simulink subsystem "cascaded_pid_controller"  (R2026a)
settings: Solver=VariableStepAuto
undefined symbols (not defined in the file): DiscIntNeverNeededParam, dspblkCoreblockFVToolHelper, FF_maneuvers, gcbh, I, P, RSFF_maneuvers, S, T
libraries: slpidlib x3, simulink x1
PreSaveFcn:
  | defaultToFileBlockNames(bdroot);
settings Model: Creator=kjhaydon  LastModifiedBy=kjhaydon

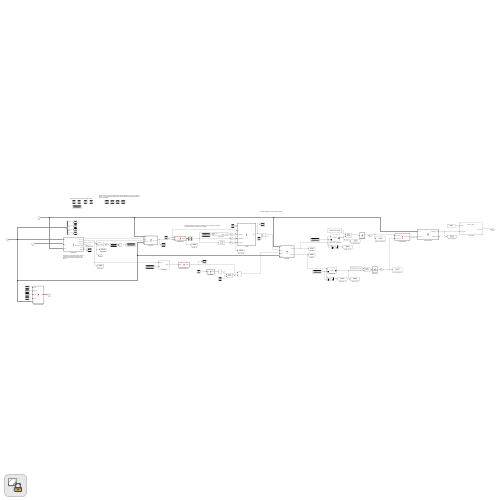
[thumbnail: Simulink's stored preview of the top-level diagram]
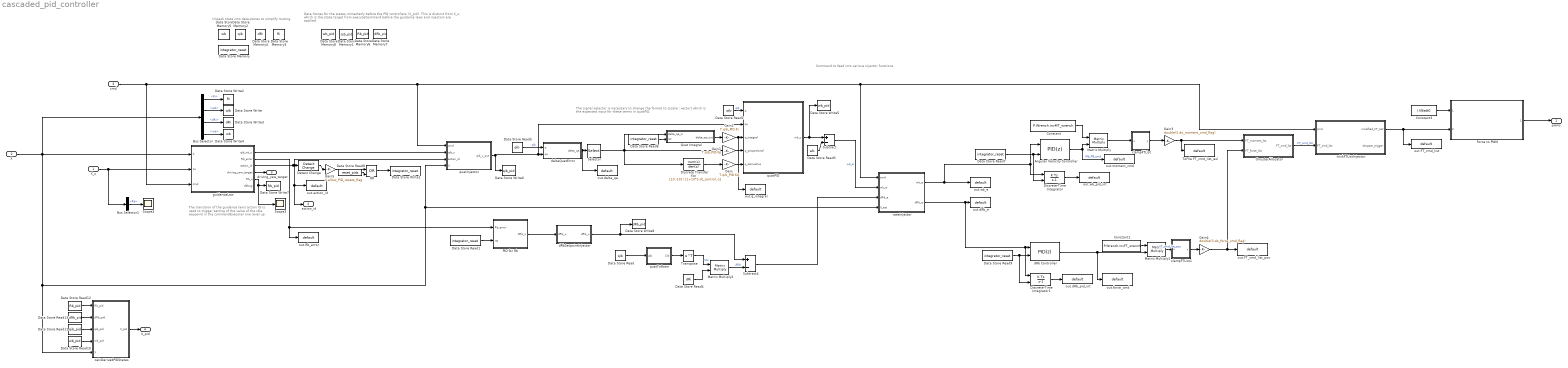
== system cascaded_pid_controller ==
  note: Data Stores for the states immediatly before the PID controllers (X_pid). This is distinct from X_u, which is the state target from executeCommand before the guidance laws and injectors are applied.
  note: Unpack state into data-stores to simplify routing.
  note: The transition of the guidance law's action ID is used to trigger setting of the value of the idle waypoint in the commandExecuter one level up.
  note: The signal selector is necessary to change the format to [scalar; vector] which
      | is the expected input for these terms in quatPID.
  note: Command to feed into various injector functions.
  X_u : Inport  SampleTime=S.dt_control
  X : Inport  Port=2  SampleTime=S.dt_control
  cmd : Inport  Port=3  SampleTime=S.dt_control
  Angular Velocity Controller : slpidlib/PID Controller  Controller=PID  Form=Parallel  TimeDomain=Discrete-time  UseExternalTs=off  SampleTime=-1  IntegratorMethod=Forward Euler  FilterMethod=Forward Euler  ControllerParametersSource=internal  P=T.wb_PID.Kp  I=T.wb_PID.Ki  UseKiTs=off  D=T.wb_PID.Kd  UseExternalDerivativeSource=off  N=T.wb_PID.N  UseFilter=on  TunerSelectOption=Transfer Function Based (PID Tuner App)  InitialConditionSource=internal  InitialConditionForIntegrator=0  InitialConditionForFilter=0  DifferentiatorICPrevScaledInput=0  ExternalReset=rising  TrackingMode=off  Kt=1  LimitOutput=on  SatLimitsSource=internal  UpperSaturationLimit=T.wb_PID.output_sat  LowerSaturationLimit=-T.wb_PID.output_sat  LinearizeAsGain=on  AntiWindupMode=clamping  Kb=1  LimitIntegrator=on  UpperIntegratorSaturationLimit=T.wb_PID.int_sat  LowerIntegratorSaturationLimit=-T.wb_PID.int_sat  POutMin=[]  POutMax=[]  IOutMin=[]  IOutMax=[]  DOutMin=[]  DOutMax=[]  NOutMin=[]  NOutMax=[]  SumOutMin=[]  SumOutMax=[]  SaturationOutMin=[]  SaturationOutMax=[]  PParamMin=[]  PParamMax=[]  IParamMin=[]  IParamMax=[]  DParamMin=[]  DParamMax=[]  NParamMin=[]  NParamMax=[]  KbParamMin=[]  KbParamMax=[]  KtParamMin=[]  KtParamMax=[]  KbOutMin=[]  KbOutMax=[]  KtOutMin=[]  KtOutMax=[]  IntegratorOutMin=[]  IntegratorOutMax=[]  FilterOutMin=[]  FilterOutMax=[]  SumI1OutMin=[]  SumI1OutMax=[]  SumI2OutMin=[]  SumI2OutMax=[]  SumI3OutMin=[]  SumI3OutMax=[]  SumI4OutMin=[]  SumI4OutMax=[]  SumDOutMin=[]  SumDOutMax=[]  DifferentiatorOutMin=[]  DifferentiatorOutMax=[]  FilterDiffOutCoefMin=[]  FilterDiffOutCoefMax=[]  ReciprocalOutMin=[]  ReciprocalOutMax=[]  SumDenOutMin=[]  SumDenOutMax=[]  SumNumOutMin=[]  SumNumOutMax=[]  DivideOutMin=[]  DivideOutMax=[]  UdiffTsProdOutMin=[]  UdiffTsProdOutMax=[]  NTsProdOutMin=[]  NTsProdOutMax=[]  UintegralTsProdOutMin=[]  UintegralTsProdOutMax=[]  UngainTsProdOutMin=[]  UngainTsProdOutMax=[]  ClampingZeroOutDataTypeStr=Inherit: Inherit via back propagation  ClampingZeroOutMin=[]  ClampingZeroOutMax=[]  FilterDenConstantOutDataTypeStr=Inherit: Inherit via back propagation  FilterDenConstantOutMin=[]  FilterDenConstantOutMax=[]  PCopyOutDataTypeStr=Inherit: Inherit via back propagation  PCopyOutMin=[]  PCopyOutMax=[]  NCopyOutDataTypeStr=Inherit: Inherit via back propagation  NCopyOutMin=[]  NCopyOutMax=[]  IntegratorContinuousStateAttributes=''  IntegratorStateMustResolveToSignalObject=off  IntegratorRTWStateStorageClass=Auto  FilterContinuousStateAttributes=''  FilterStateMustResolveToSignalObject=off  FilterRTWStateStorageClass=Auto  ParallelPVariant=InternalParameters  IdealPVariant=Disabled  IVariant=InternalParameters  DVariant=InternalParameters  IntegratorVariant=Discrete  SatVariant=Enabled  AWVariant=DiscClampingParallel  PCopyVariant=Disabled  TRVariant=Disabled  FdbkBlocksVariant=Forward  IdealPFdbkVariant=Disabled  SatFdbkVariant=Disabled  DerivativeFilterVariant=ForwardEulerFilter  NVariant=InternalParameters  NCopyVariant=Disabled  FilterICVariant=InternalICsFilter  IntegratorICVariant=InternalICs  ExternalResetVariant=ExternalReset  TRSumVariant=Passthrough  SumFdbkVariant=Disabled  SumVariant=Sum_PID  TsampFilterVariant=InternalTs  TsampNgainVariant=Passthrough  TsampIntegralVariant=Disabled_SignalSpec  ExternalSaturationOutDataTypeStr=Inherit: Same as second input  DerivativeSourceVariant=ErrorSignal  PreIntVariant=InternalPreInt
  Bus Selector : BusSelector  OutputSignals=Ri,qib,dRi,wb
  Bus Selector1 : BusSelector  OutputSignals=Rb
  Constant : Constant  Value=P.Wrench.invMT_wrench
  Constant1 : Constant  Value=P.Wrench.invFT_wrench
  Constant3 : Constant  Value=I.VBatt0
  Data Store Memory : DataStoreMemory  DataStoreName=integrator_reset  WriteAfterWriteMsg=warning  ShowAdditionalParam=off
  Data Store Memory1 : DataStoreMemory  DataStoreName=qib_pid  WriteAfterWriteMsg=warning  InitialValue=[0 0 0 1]'  ShowAdditionalParam=off
  Data Store Memory2 : DataStoreMemory  DataStoreName=qib  WriteAfterWriteMsg=warning  InitialValue=[0 0 0 1]'  ShowAdditionalParam=off
  Data Store Memory3 : DataStoreMemory  DataStoreName=Ri  WriteAfterWriteMsg=warning  InitialValue=[0 0 0]'  ShowAdditionalParam=off
  Data Store Memory4 : DataStoreMemory  DataStoreName=dRi  WriteAfterWriteMsg=warning  InitialValue=[0 0 0]'  ShowAdditionalParam=off
  Data Store Memory5 : DataStoreMemory  DataStoreName=wb  WriteAfterWriteMsg=warning  InitialValue=[0 0 0]'  ShowAdditionalParam=off
  Data Store Memory6 : DataStoreMemory  DataStoreName=Rb_pid  WriteAfterWriteMsg=warning  InitialValue=[0 0 0]'  ShowAdditionalParam=off
  Data Store Memory7 : DataStoreMemory  DataStoreName=dRb_pid  WriteAfterWriteMsg=warning  InitialValue=[0 0 0]'  ShowAdditionalParam=off
  Data Store Memory8 : DataStoreMemory  DataStoreName=wb_pid  WriteAfterWriteMsg=warning  InitialValue=[0 0 0]'  ShowAdditionalParam=off
  Data Store Read : DataStoreRead  DataStoreName=qib  IndexOptions=Index vector (dialog)  Indices=1  OutputSizes=1
  Data Store Read{1,6..7,9} (4 alike) : DataStoreRead  DataStoreName=integrator_reset  IndexOptions=Index vector (dialog)  Indices=1  OutputSizes=1
  Data Store Read10 : DataStoreRead  DataStoreName=wb_pid  IndexOptions=Index vector (dialog)  Indices=1  OutputSizes=1
  Data Store Read11 : DataStoreRead  DataStoreName=qib_pid  IndexOptions=Index vector (dialog)  Indices=1  OutputSizes=1
  Data Store Read12 : DataStoreRead  DataStoreName=Rb_pid  IndexOptions=Index vector (dialog)  Indices=1  OutputSizes=1
  Data Store Read13 : DataStoreRead  DataStoreName=dRb_pid  IndexOptions=Index vector (dialog)  Indices=1  OutputSizes=1
  Data Store Read2 : DataStoreRead  DataStoreName=qib  IndexOptions=Index vector (dialog)  Indices=1  OutputSizes=1
  Data Store Read3 : DataStoreRead  DataStoreName=wb  IndexOptions=Index vector (dialog)  Indices=1  OutputSizes=1
  Data Store Read4 : DataStoreRead  DataStoreName=dRi  IndexOptions=Index vector (dialog)  Indices=1  OutputSizes=1
  Data Store Read5 : DataStoreRead  DataStoreName=qib  IndexOptions=Index vector (dialog)  Indices=1  OutputSizes=1
  Data Store Read8 : DataStoreRead  DataStoreName=reset_pids  IndexOptions=Index vector (dialog)  Indices=1  OutputSizes=1
  Data Store Write : DataStoreWrite  DataStoreName=qib  IndexOptions=Index vector (dialog)  Indices=1  OutputSizes=1
  Data Store Write1 : DataStoreWrite  DataStoreName=integrator_reset  IndexOptions=Index vector (dialog)  Indices=1  OutputSizes=1
  Data Store Write2 : DataStoreWrite  DataStoreName=Ri  IndexOptions=Index vector (dialog)  Indices=1  OutputSizes=1
  Data Store Write3 : DataStoreWrite  DataStoreName=dRi  IndexOptions=Index vector (dialog)  Indices=1  OutputSizes=1
  Data Store Write4 : DataStoreWrite  DataStoreName=wb  IndexOptions=Index vector (dialog)  Indices=1  OutputSizes=1
  Data Store Write5 : DataStoreWrite  DataStoreName=wb_pid  IndexOptions=Index vector (dialog)  Indices=1  OutputSizes=1
  Data Store Write6 : DataStoreWrite  DataStoreName=qib_pid  IndexOptions=Index vector (dialog)  Indices=1  OutputSizes=1
  Data Store Write7 : DataStoreWrite  DataStoreName=Rb_pid  IndexOptions=Index vector (dialog)  Indices=1  OutputSizes=1
  Data Store Write8 : DataStoreWrite  DataStoreName=dRb_pid  IndexOptions=Index vector (dialog)  Indices=1  OutputSizes=1
  Detect Change : simulink/Logic and Bit Operations/Detect Change  vinit=0  OutDataTypeStr=boolean
  Discrete Transfer Fcn : DiscreteTransferFcn  LoadFcn=dspblkCoreblockFVToolHelper(gcbh,'load');  Numerator=[10,-10]  Denominator=[1+10*S.dt_control,-1]
      settings: CopyFcn=dspblkCoreblockFVToolHelper(gcbh,'copy');  DeleteFcn=dspblkCoreblockFVToolHelper(gcbh,'close');  ModelCloseFcn=dspblkCoreblockFVToolHelper(gcbh,'close');  PreSaveFcn=dspblkCoreblockFVToolHelper(gcbh,'presave');  PostSaveFcn=dspblkCoreblockFVToolHelper(gcbh,'postsave');  CloseFcn=dspblkCoreblockFVToolHelper(gcbh,'close');
  Discrete-Time Integrator : DiscreteIntegrator  gainval=T.wb_PID.Ki  ExternalReset=rising  InitialCondition=[0;0;0]  SampleTime=S.dt_control  LimitOutput=on  UpperSaturationLimit=T.wb_PID.int_sat  LowerSaturationLimit=-T.wb_PID.int_sat  ICPrevOutput=DiscIntNeverNeededParam  ICPrevScaledInput=DiscIntNeverNeededParam
  Discrete-Time Integrator1 : DiscreteIntegrator  gainval=T.dRb_PID.Ki  ExternalReset=rising  InitialCondition=[0;0;0]  SampleTime=S.dt_control  LimitOutput=on  UpperSaturationLimit=T.dRb_PID.int_sat  LowerSaturationLimit=-T.dRb_PID.int_sat  ICPrevOutput=DiscIntNeverNeededParam  ICPrevScaledInput=DiscIntNeverNeededParam
  Force to PWM : Subsystem  ReferencedSubsystem=force_to_pwm
  Gain : Gain  Gain=T.qib_PID.Kd
  Gain1 : Gain  Gain=T.qib_PID.Kp
  Gain2 : Gain  Gain=T.qib_PID.Ki
  Gain3 : Gain  Gain=double(S.do_moment_cmd_flag)
  Gain4 : Gain  Gain=double(S.do_force_cmd_flag)
  Gain5 : Gain  Gain=S.allow_PID_resets_flag
  Matrix Multiply : Product  Multiplication=Matrix(*)
  Matrix Multiply1 : Product  Multiplication=Matrix(*)
  Matrix Multiply3 : Product  Multiplication=Matrix(*)
  OR : Logic  Operator=OR  IconShape=distinctive  AllPortsSameDT=off  OutDataTypeStr=boolean
  PID for Rb : Subsystem
  Quat Integral : Subsystem
  Scope3 : Scope
      settings: ActiveDisplayYMinimum=-2.6644023015259384  ActiveDisplayYMaximum=2.5944913455232195  DataLoggingVariableName=ScopeData6
  Scope4 : Scope
      settings: ActiveDisplayYMinimum=-6.74848704493326  ActiveDisplayYMaximum=15.916420433675906  DataLoggingVariableName=ScopeData7
  Selector : Selector  InputPortWidth=4  IndexOptions=Index vector (dialog)  Indices=[4 1 2 3]  OutputSizes=1
  Subtract : Sum  Inputs=+-
  Subtract4 : Sum  Inputs=+-
  ToFIle FT_cmd_list_eul : ToFile  Filename=default  MatrixName=FT_cmd_list_eul  SaveFormat=Timeseries  SampleTime=S.dt_data
  Transpose : Math  Operator=transpose
  calcDerivedPIDStates : MATLAB Function  TreatAsAtomicUnit=on
  clampFTList : MATLAB Function  TreatAsAtomicUnit=on
  clampFTList1 : MATLAB Function  TreatAsAtomicUnit=on
  dRb Controller : slpidlib/PID Controller  Controller=PID  Form=Parallel  TimeDomain=Discrete-time  UseExternalTs=off  SampleTime=-1  IntegratorMethod=Forward Euler  FilterMethod=Forward Euler  ControllerParametersSource=internal  P=T.dRb_PID.Kp  I=T.dRb_PID.Ki  UseKiTs=off  D=T.dRb_PID.Kd  UseExternalDerivativeSource=off  N=T.dRb_PID.N  UseFilter=on  TunerSelectOption=Transfer Function Based (PID Tuner App)  InitialConditionSource=internal  InitialConditionForIntegrator=0  InitialConditionForFilter=0  DifferentiatorICPrevScaledInput=0  ExternalReset=rising  TrackingMode=off  Kt=1  LimitOutput=on  SatLimitsSource=internal  UpperSaturationLimit=T.dRb_PID.output_sat  LowerSaturationLimit=-T.dRb_PID.output_sat  LinearizeAsGain=on  AntiWindupMode=clamping  Kb=1  LimitIntegrator=on  UpperIntegratorSaturationLimit=T.dRb_PID.int_sat  LowerIntegratorSaturationLimit=-T.dRb_PID.int_sat  POutMin=[]  POutMax=[]  IOutMin=[]  IOutMax=[]  DOutMin=[]  DOutMax=[]  NOutMin=[]  NOutMax=[]  SumOutMin=[]  SumOutMax=[]  SaturationOutMin=[]  SaturationOutMax=[]  PParamMin=[]  PParamMax=[]  IParamMin=[]  IParamMax=[]  DParamMin=[]  DParamMax=[]  NParamMin=[]  NParamMax=[]  KbParamMin=[]  KbParamMax=[]  KtParamMin=[]  KtParamMax=[]  KbOutMin=[]  KbOutMax=[]  KtOutMin=[]  KtOutMax=[]  IntegratorOutMin=[]  IntegratorOutMax=[]  FilterOutMin=[]  FilterOutMax=[]  SumI1OutMin=[]  SumI1OutMax=[]  SumI2OutMin=[]  SumI2OutMax=[]  SumI3OutMin=[]  SumI3OutMax=[]  SumI4OutMin=[]  SumI4OutMax=[]  SumDOutMin=[]  SumDOutMax=[]  DifferentiatorOutMin=[]  DifferentiatorOutMax=[]  FilterDiffOutCoefMin=[]  FilterDiffOutCoefMax=[]  ReciprocalOutMin=[]  ReciprocalOutMax=[]  SumDenOutMin=[]  SumDenOutMax=[]  SumNumOutMin=[]  SumNumOutMax=[]  DivideOutMin=[]  DivideOutMax=[]  UdiffTsProdOutMin=[]  UdiffTsProdOutMax=[]  NTsProdOutMin=[]  NTsProdOutMax=[]  UintegralTsProdOutMin=[]  UintegralTsProdOutMax=[]  UngainTsProdOutMin=[]  UngainTsProdOutMax=[]  ClampingZeroOutDataTypeStr=Inherit: Inherit via back propagation  ClampingZeroOutMin=[]  ClampingZeroOutMax=[]  FilterDenConstantOutDataTypeStr=Inherit: Inherit via back propagation  FilterDenConstantOutMin=[]  FilterDenConstantOutMax=[]  PCopyOutDataTypeStr=Inherit: Inherit via back propagation  PCopyOutMin=[]  PCopyOutMax=[]  NCopyOutDataTypeStr=Inherit: Inherit via back propagation  NCopyOutMin=[]  NCopyOutMax=[]  IntegratorContinuousStateAttributes=''  IntegratorStateMustResolveToSignalObject=off  IntegratorRTWStateStorageClass=Auto  FilterContinuousStateAttributes=''  FilterStateMustResolveToSignalObject=off  FilterRTWStateStorageClass=Auto  ParallelPVariant=InternalParameters  IdealPVariant=Disabled  IVariant=InternalParameters  DVariant=InternalParameters  IntegratorVariant=Discrete  SatVariant=Enabled  AWVariant=DiscClampingParallel  PCopyVariant=Disabled  TRVariant=Disabled  FdbkBlocksVariant=Forward  IdealPFdbkVariant=Disabled  SatFdbkVariant=Disabled  DerivativeFilterVariant=ForwardEulerFilter  NVariant=InternalParameters  NCopyVariant=Disabled  FilterICVariant=InternalICsFilter  IntegratorICVariant=InternalICs  ExternalResetVariant=ExternalReset  TRSumVariant=Passthrough  SumFdbkVariant=Disabled  SumVariant=Sum_PID  TsampFilterVariant=InternalTs  TsampNgainVariant=Passthrough  TsampIntegralVariant=Disabled_SignalSpec  ExternalSaturationOutDataTypeStr=Inherit: Same as second input  DerivativeSourceVariant=ErrorSignal  PreIntVariant=InternalPreInt
  dRbSetpointInjector : MATLAB Function  TreatAsAtomicUnit=on
  deltaQuatError : MATLAB Function  TreatAsAtomicUnit=on
  guidanceLaw : MATLAB Function  TreatAsAtomicUnit=on
  out.FT_cmd_list : ToFile  Filename=default  MatrixName=FT_cmd_list  SaveFormat=Timeseries  SampleTime=S.dt_data
  out.FT_cmd_list_pos : ToFile  Filename=default  MatrixName=FT_cmd_list_pos  SaveFormat=Timeseries  SampleTime=S.dt_data
  out.Rb_error : ToFile  Filename=default  MatrixName=Rb_e  SaveFormat=Timeseries  SampleTime=S.dt_data
  out.action_id : ToFile  Filename=default  MatrixName=action_id  SaveFormat=Timeseries  SampleTime=S.dt_control
  out.dRb_e : ToFile  Filename=default  MatrixName=dRb_e  SaveFormat=Timeseries  SampleTime=S.dt_data
  out.dRb_pid_int : ToFile  Filename=default  MatrixName=dRb_pid_int  SaveFormat=Timeseries  SampleTime=S.dt_data
  out.delta_qe : ToFile  Filename=default  MatrixName=qib_e  SaveFormat=Timeseries  SampleTime=S.dt_data
  out.force_cmd : ToFile  Filename=default  MatrixName=force_cmd  SaveFormat=Timeseries  SampleTime=S.dt_data
  out.moment_cmd : ToFile  Filename=default  MatrixName=moment_cmd  SaveFormat=Timeseries  SampleTime=S.dt_data
  out.q_integral : ToFile  Filename=default  MatrixName=qib_integrator  SaveFormat=Timeseries  SampleTime=S.dt_data
  out.wb_e : ToFile  Filename=default  MatrixName=wb_e  SaveFormat=Timeseries  SampleTime=S.dt_data
  out.wb_pid_int : ToFile  Filename=default  MatrixName=wb_pid_int  SaveFormat=Timeseries  SampleTime=S.dt_data
  quatInjector : MATLAB Function  TreatAsAtomicUnit=on
  quatPID : MATLAB Function  TreatAsAtomicUnit=on
  quatToRotm : MATLAB Function  TreatAsAtomicUnit=on
  rateInjector : MATLAB Function  TreatAsAtomicUnit=on
  thrusterAllocator : MATLAB Function  TreatAsAtomicUnit=on
  trickFTListInjector : MATLAB Function  TreatAsAtomicUnit=on
  pwms : Outport
  action_id : Outport  Port=2
  driving_yaw_target : Outport  Port=3
  X_pid : Outport  Port=4
  wires:
  calcDerivedPIDStates/1(X_pid) -> X_pid/1
  dRb Controller/1 -> out.force_cmd/1, Matrix Multiply1/2
  guidanceLaw/5(Rb_u) -> Data Store Write7/1, Scope3/1
  Gain4/1 -> thrusterAllocator/2(FT_force_list), out.FT_cmd_list_pos/1
  quatInjector/1(qib_u_out) -> quatPID/2(qu), deltaQuatError/2(qu), Data Store Write6/1
  rateInjector/2(dRb_e) -> dRb Controller/1, Discrete-Time Integrator1/1, out.dRb_e/1
  Subtract4/1 -> rateInjector/3("dRb_e ")
  rateInjector/1(wb_e) -> Angular Velocity Controller/1, Discrete-Time Integrator/1, out.wb_e/1
  Subtract/1 -> rateInjector/2("wb_e ")  "wb_e"
  Data Store Read6/1 -> Quat Integral/2(rst)
  trickFTListInjector/1(modified_FT_List) -> Force to PWM/2, out.FT_cmd_list/1
  cmd/1 -> guidanceLaw/3(cmd), trickFTListInjector/1(cmd), rateInjector/1(cmd), quatInjector/1(cmd)
  thrusterAllocator/1(FT_cmd_list) -> trickFTListInjector/2(FT_cmd_list)  "FT_cmd_list"
  Force to PWM/1 -> pwms/1
  guidanceLaw/3(action_id) -> Detect Change/1, quatInjector/3(action_id), out.action_id/1, action_id/1
  guidanceLaw/1(qib_int_u) -> quatInjector/2(qib_u)
  X_u/1 -> guidanceLaw/2(Xu), Bus Selector1/1
  deltaQuatError/1(delta_qe) -> Selector/1, out.delta_qe/1
  Gain2/1 -> quatPID/3(q_integral), out.q_integral/1
  Gain1/1 -> quatPID/4(q_proportional)
  Gain/1 -> quatPID/5(q_derivative)
  quatPID/1(wb_u) -> Data Store Write5/1, Subtract/1
  Angular Velocity Controller/1 -> out.moment_cmd/1, Matrix Multiply/2  "Mb_FB_cmd"
  Constant/1 -> Matrix Multiply/1
  Constant3/1 -> Force to PWM/1
  Matrix Multiply/1 -> clampFTList/1(u)
  Constant1/1 -> Matrix Multiply1/1
  Matrix Multiply1/1 -> clampFTList1/1(u)  "FT_cmd_list_pos"
  Data Store Read/1 -> quatToRotm/1(qib)
  quatToRotm/1(Cib) -> Transpose/1
  Transpose/1 -> Matrix Multiply3/1  "Cbi"
  Matrix Multiply3/1 -> Subtract4/2  "dRb"
  Data Store Read4/1 -> Matrix Multiply3/2
  Data Store Read3/1 -> Subtract/2
  Data Store Read2/1 -> quatPID/1(q)  "qib"
  Data Store Read5/1 -> deltaQuatError/1(q)  "qib"
  Selector/1 -> Discrete Transfer Fcn/1, Gain1/1, Quat Integral/1(delta_qe_in)
  Quat Integral/1(delta_qe_out) -> Gain2/1
  Discrete Transfer Fcn/1 -> Gain/1
  guidanceLaw/2(Rb_error) -> out.Rb_error/1, PID for Rb/1(Rb_error)
  PID for Rb/1(dRb_u) -> dRbSetpointInjector/1("dRb_u ")
  guidanceLaw/4(driving_yaw_target) -> driving_yaw_target/1
  Bus Selector/1 -> Data Store Write2/1  "<Ri>"
  Bus Selector/2 -> Data Store Write/1  "<qib>"
  Bus Selector/3 -> Data Store Write3/1  "<dRi>"
  Bus Selector/4 -> Data Store Write4/1  "<wb>"
  Data Store Read7/1 -> Discrete-Time Integrator/2, Angular Velocity Controller/2
  Data Store Read9/1 -> Discrete-Time Integrator1/2, dRb Controller/2
  Discrete-Time Integrator/1 -> out.wb_pid_int/1
  Detect Change/1 -> Gain5/1
  dRbSetpointInjector/1(dRb_u) -> Data Store Write8/1, Subtract4/1
  Discrete-Time Integrator1/1 -> out.dRb_pid_int/1
  Gain3/1 -> thrusterAllocator/1(FT_moment_list), ToFIle FT_cmd_list_eul/1
  Gain5/1 -> OR/1
  OR/1 -> Data Store Write1/1
  Data Store Read8/1 -> OR/2
  Data Store Read11/1 -> calcDerivedPIDStates/3(qib_pid)
  X/1 -> guidanceLaw/1(X), Bus Selector/1, quatInjector/4(X), rateInjector/4(X_est), calcDerivedPIDStates/5(X)
  Data Store Read12/1 -> calcDerivedPIDStates/1(Rb_pid)
  Data Store Read10/1 -> calcDerivedPIDStates/4(wb_pid)
  Data Store Read13/1 -> calcDerivedPIDStates/2(dRb_pid)
  clampFTList/1(y) -> Gain3/1
  clampFTList1/1(y) -> Gain4/1
  Data Store Read1/1 -> PID for Rb/2(rst)
  Bus Selector1/1 -> Scope4/1  "<Rb>"

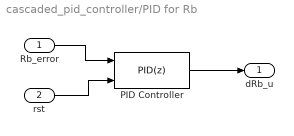
== system cascaded_pid_controller/PID for Rb ==
  Rb_error : Inport
  rst : Inport  Port=2
  PID Controller : slpidlib/PID Controller  Controller=PID  Form=Parallel  TimeDomain=Discrete-time  UseExternalTs=off  SampleTime=-1  IntegratorMethod=Forward Euler  FilterMethod=Forward Euler  ControllerParametersSource=internal  P=T.Rb_PID.Kp  I=T.Rb_PID.Ki  UseKiTs=off  D=T.Rb_PID.Kd  UseExternalDerivativeSource=off  N=T.Rb_PID.N  UseFilter=on  TunerSelectOption=Transfer Function Based (PID Tuner App)  InitialConditionSource=internal  InitialConditionForIntegrator=0  InitialConditionForFilter=0  DifferentiatorICPrevScaledInput=0  ExternalReset=rising  TrackingMode=off  Kt=1  LimitOutput=on  SatLimitsSource=internal  UpperSaturationLimit=T.Rb_PID.output_sat  LowerSaturationLimit=-T.Rb_PID.output_sat  LinearizeAsGain=on  AntiWindupMode=clamping  Kb=1  LimitIntegrator=on  UpperIntegratorSaturationLimit=T.Rb_PID.int_sat  LowerIntegratorSaturationLimit=-T.Rb_PID.int_sat  POutMin=[]  POutMax=[]  IOutMin=[]  IOutMax=[]  DOutMin=[]  DOutMax=[]  NOutMin=[]  NOutMax=[]  SumOutMin=[]  SumOutMax=[]  SaturationOutMin=[]  SaturationOutMax=[]  PParamMin=[]  PParamMax=[]  IParamMin=[]  IParamMax=[]  DParamMin=[]  DParamMax=[]  NParamMin=[]  NParamMax=[]  KbParamMin=[]  KbParamMax=[]  KtParamMin=[]  KtParamMax=[]  KbOutMin=[]  KbOutMax=[]  KtOutMin=[]  KtOutMax=[]  IntegratorOutMin=[]  IntegratorOutMax=[]  FilterOutMin=[]  FilterOutMax=[]  SumI1OutMin=[]  SumI1OutMax=[]  SumI2OutMin=[]  SumI2OutMax=[]  SumI3OutMin=[]  SumI3OutMax=[]  SumI4OutMin=[]  SumI4OutMax=[]  SumDOutMin=[]  SumDOutMax=[]  DifferentiatorOutMin=[]  DifferentiatorOutMax=[]  FilterDiffOutCoefMin=[]  FilterDiffOutCoefMax=[]  ReciprocalOutMin=[]  ReciprocalOutMax=[]  SumDenOutMin=[]  SumDenOutMax=[]  SumNumOutMin=[]  SumNumOutMax=[]  DivideOutMin=[]  DivideOutMax=[]  UdiffTsProdOutMin=[]  UdiffTsProdOutMax=[]  NTsProdOutMin=[]  NTsProdOutMax=[]  UintegralTsProdOutMin=[]  UintegralTsProdOutMax=[]  UngainTsProdOutMin=[]  UngainTsProdOutMax=[]  ClampingZeroOutDataTypeStr=Inherit: Inherit via back propagation  ClampingZeroOutMin=[]  ClampingZeroOutMax=[]  FilterDenConstantOutDataTypeStr=Inherit: Inherit via back propagation  FilterDenConstantOutMin=[]  FilterDenConstantOutMax=[]  PCopyOutDataTypeStr=Inherit: Inherit via back propagation  PCopyOutMin=[]  PCopyOutMax=[]  NCopyOutDataTypeStr=Inherit: Inherit via back propagation  NCopyOutMin=[]  NCopyOutMax=[]  IntegratorContinuousStateAttributes=''  IntegratorStateMustResolveToSignalObject=off  IntegratorRTWStateStorageClass=Auto  FilterContinuousStateAttributes=''  FilterStateMustResolveToSignalObject=off  FilterRTWStateStorageClass=Auto  ParallelPVariant=InternalParameters  IdealPVariant=Disabled  IVariant=InternalParameters  DVariant=InternalParameters  IntegratorVariant=Discrete  SatVariant=Enabled  AWVariant=DiscClampingParallel  PCopyVariant=Disabled  TRVariant=Disabled  FdbkBlocksVariant=Forward  IdealPFdbkVariant=Disabled  SatFdbkVariant=Disabled  DerivativeFilterVariant=ForwardEulerFilter  NVariant=InternalParameters  NCopyVariant=Disabled  FilterICVariant=InternalICsFilter  IntegratorICVariant=InternalICs  ExternalResetVariant=ExternalReset  TRSumVariant=Passthrough  SumFdbkVariant=Disabled  SumVariant=Sum_PID  TsampFilterVariant=InternalTs  TsampNgainVariant=Passthrough  TsampIntegralVariant=Disabled_SignalSpec  ExternalSaturationOutDataTypeStr=Inherit: Same as second input  DerivativeSourceVariant=ErrorSignal  PreIntVariant=InternalPreInt
  dRb_u : Outport
  wires:
  rst/1 -> PID Controller/2
  PID Controller/1 -> dRb_u/1
  Rb_error/1 -> PID Controller/1

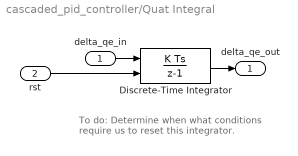
== system cascaded_pid_controller/Quat Integral ==
  note: To do: Determine when what conditions
      | require us to reset this integrator.
  delta_qe_in : Inport
  rst : Inport  Port=2
  Discrete-Time Integrator : DiscreteIntegrator  ExternalReset=rising  SampleTime=-1  LimitOutput=on  UpperSaturationLimit=T.qib_PID.int_sat  LowerSaturationLimit=-T.qib_PID.int_sat  ICPrevOutput=DiscIntNeverNeededParam  ICPrevScaledInput=DiscIntNeverNeededParam
  delta_qe_out : Outport
  wires:
  rst/1 -> Discrete-Time Integrator/2
  Discrete-Time Integrator/1 -> delta_qe_out/1
  delta_qe_in/1 -> Discrete-Time Integrator/1

== matlab function cascaded_pid_controller/quatPID ==
  data: q input; qu input; q_integral input; q_proportional input; wb_u output; q_derivative input; S parameter
function wb_u = fcn(q, qu, q_integral, q_proportional, q_derivative, S)

overwrite_rate_setpoint_flag = S.overwrite_rate_setpoint_flag;
wb_sp_inject = S.wb_sp_inject;

wb_u = quatPID(q, qu, q_proportional, q_integral, q_derivative, overwrite_rate_setpoint_flag, wb_sp_inject);

== matlab function cascaded_pid_controller/quatToRotm ==
  data: qib input; Cib output
function Cib = fcn(qib)

Cib = quatToRotm(qib);

== matlab function cascaded_pid_controller/rateInjector ==
  data: cmd input Bus: cmd_bus; wb_e input; wb_e output; dRb_e input; dRb_e output; RSFF_maneuvers parameter Bus: RSFF_maneuver_bus; X_est input Bus: X_bus; S parameter
function [wb_e, dRb_e] = fcn(cmd, wb_e, dRb_e, RSFF_maneuvers, X_est, S)

overwrite_rate_error_flag = S.overwrite_rate_error_flag;
wb_error_inject = S.wb_error_inject;
dRb_error_inject = S.dRb_error_inject;

[wb_e, dRb_e] = rateInjector(cmd, wb_e, dRb_e, X_est, RSFF_maneuvers, overwrite_rate_error_flag, wb_error_inject, dRb_error_inject);

== matlab function cascaded_pid_controller/thrusterAllocator ==
  data: FT_moment_list input; FT_cmd_list output; FT_force_list input; P parameter
function FT_cmd_list = fcn(FT_moment_list, FT_force_list, P)

max_thruster_force = P.Constants.max_thruster_force;

FT_cmd_list = thrusterAllocator(FT_moment_list, FT_force_list, max_thruster_force);

== matlab function cascaded_pid_controller/trickFTListInjector ==
  data: cmd input; modified_FT_List output size=[8,1]; FT_cmd_list input; FF_maneuvers parameter Bus: FF_maneuvers_bus; S parameter; dropper_trigger output
function [modified_FT_List, dropper_trigger] = fcn(cmd, FT_cmd_list, FF_maneuvers,S)

overwrite_FT_list_flag = S.overwrite_FT_list_flag;
FT_list_inject = S.FT_list_inject;

[modified_FT_List, dropper_trigger] = trickFTListInjector(cmd, FT_cmd_list, FF_maneuvers, overwrite_FT_list_flag, FT_list_inject);

== matlab function cascaded_pid_controller/clampFTList ==
  data: u input; y output; P parameter
function y = fcn(u, P)

max_thruster_force = P.Constants.max_thruster_force;

y = max(-max_thruster_force, min(max_thruster_force, u));

== matlab function cascaded_pid_controller/clampFTList1 ==
  data: u input; y output; P parameter
function y = fcn(u, P)

max_thruster_force = P.Constants.max_thruster_force;

y = max(-max_thruster_force, min(max_thruster_force, u));

== matlab function cascaded_pid_controller/calcDerivedPIDStates ==
  data: Rb_pid input; X_pid output Bus: X_bus; dRb_pid input; qib_pid input; wb_pid input; X input Bus: X_bus
function X_pid = fcn(Rb_pid, dRb_pid, qib_pid, wb_pid, X)

X_pid = calcDerivedPIDStates(Rb_pid, dRb_pid, qib_pid, wb_pid, X);

== matlab function cascaded_pid_controller/dRbSetpointInjector ==
  data: dRb_u input; dRb_u output; S parameter
function dRb_u=fcn(dRb_u, S)

dRb_sp_inject = S.dRb_sp_inject;
overwrite_rate_setpoint_flag = S.overwrite_rate_setpoint_flag;

if(overwrite_rate_setpoint_flag)
    dRb_u = dRb_sp_inject;
end

== matlab function cascaded_pid_controller/deltaQuatError ==
  data: q input; delta_qe output; qu input; S parameter
function delta_qe = fcn(q, qu, S)

overwrite_state_error_flag = S.overwrite_state_error_flag;
eul_error_inject = S.eul_error_inject;

delta_qe = deltaQuatError(q, qu, overwrite_state_error_flag, eul_error_inject);

== matlab function cascaded_pid_controller/guidanceLaw ==
  settings: updateMethod=DISCRETE  sampleTime=S.dt_control
  data: X input Bus: X_bus; qib_int_u output; Xu input; cmd input Bus: cmd_bus; Rb_error output; T parameter; action_id output; driving_yaw_target output; Rb_u output; debug output; S parameter
function [qib_int_u, Rb_error, action_id, driving_yaw_target, Rb_u,debug] = fcn(X, Xu, cmd, T, S)

Ri_e_tol = T.Ri_e_tol;
Eul_e_tol = T.Eul_e_tol;
overwrite_state_error_flag = S.overwrite_state_error_flag;
Rb_error_inject = S.Rb_error_inject;
overwrite_state_setpoint_flag = S.overwrite_state_setpoint_flag;
Rb_sp_inject = S.Rb_sp_inject;

[qib_int_u, Rb_error, action_id, driving_yaw_target, Rb_u,debug] = guidanceLaw(X, Xu, Ri_e_tol, Eul_e_tol, cmd, overwrite_state_error_flag, Rb_error_inject, overwrite_state_setpoint_flag, Rb_sp_inject);

== matlab function cascaded_pid_controller/quatInjector ==
  data: cmd input; qib_u_out output size=[4 1]; qib_u input; action_id input; X input; S parameter
function qib_u_out  = fcn(cmd, qib_u, action_id, X, S)

eul_sp_inject = S.eul_sp_inject;
overwrite_state_setpoint_flag = S.overwrite_state_setpoint_flag;

qib_u_out = quatInjector(cmd, qib_u, action_id, X, eul_sp_inject, overwrite_state_setpoint_flag);
